simulink model "Plant_blockdiagram"  (R2025b)
settings: Solver=VariableStepAuto  StartTime=0.0  StopTime=20  RelTol=1e-3
PreLoadFcn:
  | [~, p] = plant_model(1, 0.99, 0.018, 0.0106); kv = p.kv; R = p.R; L = p.L; ki = p.ki; kb = p.kb; N = p.N; eta = p.eta; Me = p.Me; ks = p.ks; bs = p.bs; ml = p.ml; tauS = p.tauS;
InitFcn:
  | [~, p] = plant_model(1, 0.99, 0.018, 0.0106); kv = p.kv; R = p.R; L = p.L; ki = p.ki; kb = p.kb; N = p.N; eta = p.eta; Me = p.Me; ks = p.ks; bs = p.bs; ml = p.ml; tauS = p.tauS;
settings Model: Creator=havard  LastModifiedBy=havard

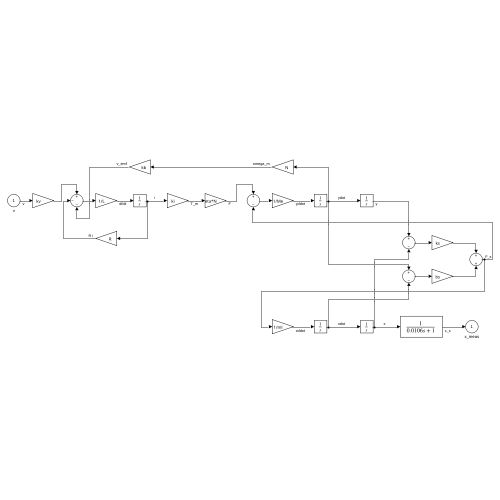
[thumbnail: Simulink's stored preview of the top-level diagram]
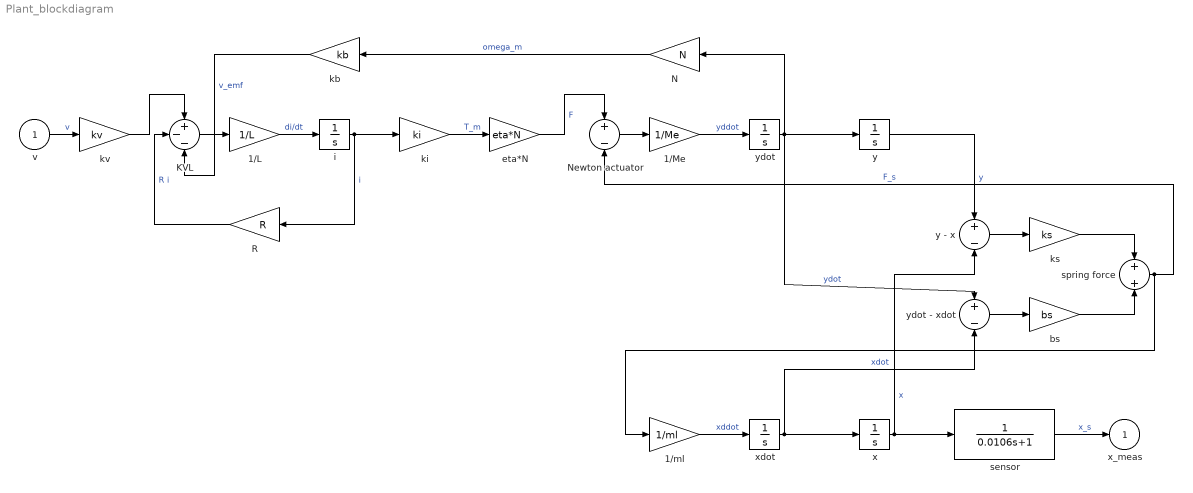
== system Plant_blockdiagram ==
  v : Inport
  1/L : Gain  Gain=1/L
  1/Me : Gain  Gain=1/Me
  1/ml : Gain  Gain=1/ml
  KVL : Sum  Inputs=+--
  N : Gain  Gain=N
  Newton actuator : Sum  Inputs=+-
  R : Gain  Gain=R
  bs : Gain  Gain=bs
  eta*N : Gain  Gain=eta*N
  i : Integrator
  kb : Gain  Gain=kb
  ki : Gain  Gain=ki
  ks : Gain  Gain=ks
  kv : Gain  Gain=kv
  sensor : TransferFcn  Numerator=1  Denominator=[0.0106 1]
  spring force : Sum
  x : Integrator
  xdot : Integrator
  y : Integrator
  y - x : Sum  Inputs=+-
  ydot : Integrator
  ydot - xdot : Sum  Inputs=+-
  x_meas : Outport
  wires:
  v/1 -> kv/1  "v"
  kv/1 -> KVL/1
  KVL/1 -> 1/L/1
  1/L/1 -> i/1  "di/dt"
  i/1 -> ki/1, R/1  "i"
  ki/1 -> eta*N/1  "T_m"
  eta*N/1 -> Newton actuator/1  "F"
  Newton actuator/1 -> 1/Me/1
  1/Me/1 -> ydot/1  "yddot"
  ydot/1 -> y/1, N/1, ydot - xdot/1  "ydot"
  R/1 -> KVL/2  "R i"
  N/1 -> kb/1  "omega_m"
  kb/1 -> KVL/3  "v_emf"
  xdot/1 -> x/1, ydot - xdot/2  "xdot"
  x/1 -> sensor/1, y - x/2  "x"
  y/1 -> y - x/1  "y"
  y - x/1 -> ks/1
  ydot - xdot/1 -> bs/1
  ks/1 -> spring force/1
  bs/1 -> spring force/2
  spring force/1 -> Newton actuator/2, 1/ml/1  "F_s"
  1/ml/1 -> xdot/1  "xddot"
  sensor/1 -> x_meas/1  "x_s"
